simulink library "Lib_Piccolo"  (R2018b)
settings: Solver=VariableStepAuto  StartTime=0.0  StopTime=10.0  RelTol=1e-3
values from neighbouring files (symbols this model uses):
  AccelErrInt2Brakes = 0.15    [SimulationControlConfig16P.m]    (also in SimulationControlConfig16P_LEGACY.m; SimulationControlConfigTAILLESS.m = 0.2; SimulationControlConfigUTAIL.m = 0.2)
  AileronMax = 25    [SimulationControlConfig16P.m]    (also in SimulationControlConfig16P_LEGACY.m; SimulationControlConfigTAILLESS.m; SimulationControlConfigUTAIL.m)
  AileronPower = 0.00268    [SimulationControlConfig16P.m]    (also in SimulationControlConfig16P_LEGACY.m; SimulationControlConfigTAILLESS.m; SimulationControlConfigUTAIL.m)
  AileronSurfaceMax = 45    [SimulationControlConfig16P.m]    (also in SimulationControlConfig16P_LEGACY.m)
  AileronTrim = 0    [SimulationControlConfig16P.m]    (also in SimulationControlConfig16P_LEGACY.m; SimulationControlConfigTAILLESS.m; SimulationControlConfigUTAIL.m)
  Alt = 1000 + TerrainHeight    [SimulationStateConfig.m]
  AltCruise_m = testPlans(testIndx).terrainElevation * 0.3048 + 200    [SimulationControlConfig16P.m]    (also in SimulationControlConfigTAILLESS.m = 1083; SimulationControlConfigUTAIL.m = testPlans(testIndx).terrainElevation * 0.3048 + 152)
  AltitudeRate2PitchCmdIntegratorInit = 0.1    [SimulationControlPre.m]
  AltMax = 10000    [SimulationControlConfig16P.m]    (also in SimulationControlConfig16P_LEGACY.m; SimulationControlConfigTAILLESS.m; SimulationControlConfigUTAIL.m)
  AltMaxAccel = 1.25    [SimulationControlConfig16P.m]    (also in SimulationControlConfig16P_LEGACY.m = 0.9; SimulationControlConfigTAILLESS.m = 1.7; SimulationControlConfigUTAIL.m = 2)
  AltMin = 0    [SimulationControlConfig16P.m]    (also in SimulationControlConfig16P_LEGACY.m; SimulationControlConfigTAILLESS.m; SimulationControlConfigUTAIL.m)
  AltRateCmd2Pitch = 0.50    (= 0.5)    [SimulationControlConfig16P.m]    (also in SimulationControlConfig16P_LEGACY.m = 0.6; SimulationControlConfigTAILLESS.m = 0.2; SimulationControlConfigUTAIL.m = 0.3)
  AltRateError2Pitch = 0.40    (= 0.4)    [SimulationControlConfig16P.m]    (also in SimulationControlConfig16P_LEGACY.m; SimulationControlConfigTAILLESS.m = 0.55; SimulationControlConfigUTAIL.m = 0.55)
  AltRateErrorInt2Pitch = 0.50    (= 0.5)    [SimulationControlConfig16P.m]    (also in SimulationControlConfig16P_LEGACY.m = 0.45; SimulationControlConfigTAILLESS.m; SimulationControlConfigUTAIL.m = 0.75)
  AltRateLpfCutOff = 3    [SimulationControlConfig16P.m]    (also in SimulationControlConfig16P_LEGACY.m; SimulationControlConfigTAILLESS.m = 2; SimulationControlConfigUTAIL.m = 2)
  AutoNosegear2Rudder = 26    [SimulationControlConfig16P.m]    (also in SimulationControlConfig16P_LEGACY.m; SimulationControlConfigTAILLESS.m = 25.2; SimulationControlConfigUTAIL.m = 14)
  b = 5.54    [SimulationControlConfig16P.m]    (also in SimulationControlConfig16P_LEGACY.m; SimulationControlConfigTAILLESS.m = 2.37; SimulationControlConfigUTAIL.m = 2.37)
  Bank2AileronIntegratorInit = 0    [SimulationControlPre.m]
  BankMax_User = BankMax_User/180*pi    (= 0.523598775598)    [SimulationControlConfig16P.m]    (also in SimulationControlConfig16P_LEGACY.m; SimulationControlConfigTAILLESS.m = 0.610865238198; SimulationControlConfigUTAIL.m = 0.628318530718)
  baseLegFlaps = 20    [SimulationControlConfig16P.m]    (also in SimulationControlConfig16P_LEGACY.m = 0; SimulationControlConfigTAILLESS.m = 15; SimulationControlConfigUTAIL.m = 10)
  C = GeneticOpt.C    [SimulationCostFunction.m]
  c = Sw/b    (= 0.841696750903)    [SimulationControlConfig16P.m]    (also in SimulationControlConfig16P_LEGACY.m; SimulationControlConfigTAILLESS.m = 0.354008438819; SimulationControlConfigUTAIL.m = 0.354008438819)
  cell2WheelFactorMG = 5.98    [SimulationSensorConfig16P_LEGACY.m]
  cell2WheelFactorNG = 1    [SimulationSensorConfig16P_LEGACY.m]
  cellSatMaxMG = 15000    [SimulationSensorConfig16P.m]    (also in SimulationSensorConfig16P_LEGACY.m; SimulationSensorConfigTAILLESS7P.m; SimulationSensorConfigUTAIL7P.m)
  cellSatMaxNG = 1000    [SimulationSensorConfig16P.m]    (also in SimulationSensorConfig16P_LEGACY.m; SimulationSensorConfigTAILLESS7P.m; SimulationSensorConfigUTAIL7P.m)
  cellSatMinMG = -15000    [SimulationSensorConfig16P.m]    (also in SimulationSensorConfig16P_LEGACY.m; SimulationSensorConfigTAILLESS7P.m; SimulationSensorConfigUTAIL7P.m)
  cellSatMinNG = -1000    [SimulationSensorConfig16P.m]    (also in SimulationSensorConfig16P_LEGACY.m; SimulationSensorConfigTAILLESS7P.m; SimulationSensorConfigUTAIL7P.m)
  CL_Limit = CL_Max    (= 0.54)    [SimulationControlConfig16P.m]    (also in SimulationControlConfig16P_LEGACY.m; SimulationControlConfigTAILLESS.m; SimulationControlConfigUTAIL.m = 0.53)
  CL_Max = 0.54    [SimulationControlConfig16P.m]    (also in SimulationControlConfig16P_LEGACY.m; SimulationControlConfigTAILLESS.m; SimulationControlConfigUTAIL.m = 0.53)
  CL_Max_Nom = 0.465    [SimulationControlConfig16P.m]    (also in SimulationControlConfig16P_LEGACY.m; SimulationControlConfigTAILLESS.m = 0.39; SimulationControlConfigUTAIL.m)
  CL_Min = 0    [SimulationControlConfig16P.m]    (also in SimulationControlConfig16P_LEGACY.m; SimulationControlConfigTAILLESS.m; SimulationControlConfigUTAIL.m)
  ClimbMaxFraction = 0.35    [SimulationControlConfig16P.m]    (also in SimulationControlConfig16P_LEGACY.m = 0.24; SimulationControlConfigTAILLESS.m = 0.19; SimulationControlConfigUTAIL.m = 0.21)
  ClimboutMaxBank = 7.0    (= 7)    [SimulationControlConfig16P.m]    (also in SimulationControlConfig16P_LEGACY.m; SimulationControlConfigTAILLESS.m = 5; SimulationControlConfigUTAIL.m)
  ClimboutTimer = 7.0    (= 7)    [SimulationControlConfig16P.m]    (also in SimulationControlConfig16P_LEGACY.m; SimulationControlConfigTAILLESS.m; SimulationControlConfigUTAIL.m)
  dCl_per_dFlap = 0.005581818    [SimulationControlConfig16P.m]    (also in SimulationControlConfig16P_LEGACY.m = 0; SimulationControlConfigTAILLESS.m = 0; SimulationControlConfigUTAIL.m = 0)
  DecelerationCmd = 3.1    [SimulationControlConfig16P.m]    (also in SimulationControlConfig16P_LEGACY.m; SimulationControlConfigTAILLESS.m = 0.1; SimulationControlConfigUTAIL.m = 0.1)
  DeRotateLogicEndTimer = abs((NoseDownLimit_Deg-1)/DeRotateRamp_Dps)    [SimulationControlConfig16P.m]    (also in SimulationControlConfig16P_LEGACY.m; SimulationControlConfigTAILLESS.m; SimulationControlConfigUTAIL.m)
  DeRotateLogicHoldNoseUpTimer = 0.1    [SimulationControlConfig16P.m]    (also in SimulationControlConfig16P_LEGACY.m; SimulationControlConfigTAILLESS.m; SimulationControlConfigUTAIL.m)
  DeRotateLogicTimerTimeout = 2    [SimulationControlConfig16P.m]    (also in SimulationControlConfig16P_LEGACY.m; SimulationControlConfigTAILLESS.m; SimulationControlConfigUTAIL.m)
  DeRotateLowerCmdSaturation = 0    [SimulationControlConfig16P.m]    (also in SimulationControlConfig16P_LEGACY.m; SimulationControlConfigTAILLESS.m; SimulationControlConfigUTAIL.m)
  DeRotateRamp_Dps = 3    [SimulationControlConfig16P.m]    (also in SimulationControlConfig16P_LEGACY.m; SimulationControlConfigTAILLESS.m = 8; SimulationControlConfigUTAIL.m = 8)
  DeRotateUpperCmdSaturation = 7    [SimulationControlConfig16P.m]    (also in SimulationControlConfig16P_LEGACY.m; SimulationControlConfigTAILLESS.m; SimulationControlConfigUTAIL.m)
  DescentMaxFraction = 0.22    [SimulationControlConfig16P.m]    (also in SimulationControlConfig16P_LEGACY.m = 0.2; SimulationControlConfigTAILLESS.m = 0.17; SimulationControlConfigUTAIL.m = 0.17)
  DesktopSimTerrainOffset_m = 0.406    [SimulationAircraftConfig.m]
  downwindFlaps = 0    [SimulationControlConfig16P.m]    (also in SimulationControlConfig16P_LEGACY.m; SimulationControlConfigTAILLESS.m; SimulationControlConfigUTAIL.m)
  DP_init = 0.5*1.225*V_init^2    [SimulationControlConfig16P.m]    (also in SimulationControlConfig16P_LEGACY.m; SimulationControlConfigTAILLESS.m; SimulationControlConfigUTAIL.m)
  dscNoiseMG = 1    [SimulationSensorConfig16P_LEGACY.m]
  dscNoiseNG = 0.25    [SimulationSensorConfig16P_LEGACY.m]
  DSCnumBits = 24    [SimulationSensorConfig16P.m]    (also in SimulationSensorConfig16P_LEGACY.m; SimulationSensorConfigTAILLESS7P.m; SimulationSensorConfigUTAIL7P.m)
  DSCRangeMaxMG = 15000    [SimulationSensorConfig16P.m]    (also in SimulationSensorConfig16P_LEGACY.m; SimulationSensorConfigTAILLESS7P.m; SimulationSensorConfigUTAIL7P.m)
  DSCRangeMaxNG = 1000    [SimulationSensorConfig16P.m]    (also in SimulationSensorConfig16P_LEGACY.m; SimulationSensorConfigTAILLESS7P.m; SimulationSensorConfigUTAIL7P.m)
  DSCRangeMinMG = -15000    [SimulationSensorConfig16P.m]    (also in SimulationSensorConfig16P_LEGACY.m; SimulationSensorConfigTAILLESS7P.m; SimulationSensorConfigUTAIL7P.m)
  DSCRangeMinNG = -1000    [SimulationSensorConfig16P.m]    (also in SimulationSensorConfig16P_LEGACY.m; SimulationSensorConfigTAILLESS7P.m; SimulationSensorConfigUTAIL7P.m)
  dt = DLLSim.dt    [SimulationTimeStep.m]    (also in SimulationTrim.m = 0.02)
  EarlyTouchdownThreshold = 3.0    (= 3)    [SimulationControlConfig16P.m]    (also in SimulationControlConfig16P_LEGACY.m; SimulationControlConfigTAILLESS.m = 2.2; SimulationControlConfigUTAIL.m = 2.5)
  ElevatorDeflectionRate = 15    [SimulationControlConfig16P.m]    (also in SimulationControlConfig16P_LEGACY.m = 12; SimulationControlConfigTAILLESS.m = 10; SimulationControlConfigUTAIL.m = 12)
  ElevatorMax = 25    [SimulationControlConfig16P.m]    (also in SimulationControlConfig16P_LEGACY.m; SimulationControlConfigTAILLESS.m; SimulationControlConfigUTAIL.m)
  ElevatorPower = -0.002209    [SimulationControlConfig16P.m]    (also in SimulationControlConfig16P_LEGACY.m; SimulationControlConfigTAILLESS.m = -0.002956; SimulationControlConfigUTAIL.m = -0.00205983)
  ElevatorTrim = -3.5    [SimulationControlConfig16P.m]    (also in SimulationControlConfig16P_LEGACY.m; SimulationControlConfigTAILLESS.m = -6; SimulationControlConfigUTAIL.m = -8)
  elevonBias = 0    [SimulationControlConfig16P.m]    (also in SimulationControlConfig16P_LEGACY.m; SimulationControlConfigTAILLESS.m; SimulationControlConfigUTAIL.m)
  Enable_TAS_Protection = 0    [SimulationControlConfig16P.m]    (also in SimulationControlConfig16P_LEGACY.m; SimulationControlConfigTAILLESS.m; SimulationControlConfigUTAIL.m)
  EnableCrossTrackAbort = 1    [SimulationControlConfig16P.m]    (also in SimulationControlConfigTAILLESS.m; SimulationControlConfigUTAIL.m)
  EnergyBandwidth = 0.02    [SimulationControlConfig16P.m]    (also in SimulationControlConfig16P_LEGACY.m; SimulationControlConfigTAILLESS.m = 0.06; SimulationControlConfigUTAIL.m = 0.06)
  EngineLhFuelCut = 0    [SimulationAircraftConfig.m]
  EngineRhFuelCut = 0    [SimulationAircraftConfig.m]
  FastThrottleRate = 0.075    [SimulationControlConfig16P.m]    (also in SimulationControlConfig16P_LEGACY.m = 0.05; SimulationControlConfigTAILLESS.m = 0.1; SimulationControlConfigUTAIL.m = 0.1)
  FilterWarmUpTime = 2    [SimulationSensorConfig16P.m]    (also in SimulationSensorConfig16P_LEGACY.m; SimulationSensorConfigTAILLESS7P.m; SimulationSensorConfigUTAIL7P.m)
  finalApproachFlaps = 20    [SimulationControlConfig16P.m]    (also in SimulationControlConfig16P_LEGACY.m = 0; SimulationControlConfigTAILLESS.m = 22; SimulationControlConfigUTAIL.m = 10)
  FinalDescentSlope_Deg = testPlans(testIndx).descentSlope    [SimulationControlConfig16P.m]    (also in SimulationControlConfig16P_LEGACY.m; SimulationControlConfigTAILLESS.m; SimulationControlConfigUTAIL.m)
  flapMax = 0    [SimulationControlConfig16P.m]    (also in SimulationControlConfig16P_LEGACY.m; SimulationControlConfigTAILLESS.m; SimulationControlConfigUTAIL.m)
  flapRate = 7.5    [SimulationControlConfig16P.m]    (also in SimulationControlConfig16P_LEGACY.m; SimulationControlConfigTAILLESS.m = 6.6; SimulationControlConfigUTAIL.m)
  FlareHeight = 5    [SimulationControlConfig16P.m]    (also in SimulationControlConfig16P_LEGACY.m = 4.8; SimulationControlConfigTAILLESS.m = 2.5; SimulationControlConfigUTAIL.m = 2)
  FlareVerticalRate_mps = -0.4    [SimulationControlConfig16P.m]    (also in SimulationControlConfig16P_LEGACY.m = -0.5; SimulationControlConfigTAILLESS.m = -0.15; SimulationControlConfigUTAIL.m = -0.15)
  Fp_Aileron = 0.55*2*pi*RollRateLpfCutoff*dt    [SimulationControlConfig16P.m]    (also in SimulationControlConfig16P_LEGACY.m; SimulationControlConfigTAILLESS.m; SimulationControlConfigUTAIL.m)
  Fp_Alt = 0.55*AltBandwidth    (= 0.099)    [SimulationControlConfig16P.m]    (also in SimulationControlConfig16P_LEGACY.m; SimulationControlConfigTAILLESS.m = 0.587477826221; SimulationControlConfigUTAIL.m = 0.69115038379)
  Fp_AltRate = 0.55*2*pi*AltRateLpfCutOff*dt    [SimulationControlConfig16P.m]    (also in SimulationControlConfig16P_LEGACY.m; SimulationControlConfigTAILLESS.m; SimulationControlConfigUTAIL.m)
  Fp_Elevator = 0.55*2*pi*PitchRateLpfCutoff*dt    [SimulationControlConfig16P.m]    (also in SimulationControlConfig16P_LEGACY.m; SimulationControlConfigTAILLESS.m; SimulationControlConfigUTAIL.m)
  Fp_Energy = 0.55*2*pi*EnergyBandwidth    (= 0.069115038379)    [SimulationControlConfig16P.m]    (also in SimulationControlConfig16P_LEGACY.m; SimulationControlConfigTAILLESS.m = 0.207345115137; SimulationControlConfigUTAIL.m = 0.207345115137)
  Fp_Energy2 = 0.55*2*pi*EnergyBandwidth*dt    [SimulationControlConfig16P.m]    (also in SimulationControlConfig16P_LEGACY.m; SimulationControlConfigTAILLESS.m; SimulationControlConfigUTAIL.m)
  Fp_Pitch = 0.55*2*pi*PitchBandwidth    (= 2.76460153516)    [SimulationControlConfig16P.m]    (also in SimulationControlConfig16P_LEGACY.m = 3.11017672705; SimulationControlConfigTAILLESS.m = 3.80132711084; SimulationControlConfigUTAIL.m = 2.41902634326)
  Fp_Pitch_2 = 0.55*2*pi*PitchBandwidth*dt    [SimulationControlConfig16P.m]    (also in SimulationControlConfig16P_LEGACY.m; SimulationControlConfigTAILLESS.m; SimulationControlConfigUTAIL.m)
  Fp_Roll = RollBandwidth^2    (= 1)    [SimulationControlConfig16P.m]    (also in SimulationControlConfig16P_LEGACY.m = 1.44; SimulationControlConfigTAILLESS.m; SimulationControlConfigUTAIL.m)
  Fp_Rudder = 0.55*2*pi*YawRateLpfCutoff*dt    [SimulationControlConfig16P.m]    (also in SimulationControlConfig16P_LEGACY.m; SimulationControlConfigTAILLESS.m; SimulationControlConfigUTAIL.m)
  Fp_TAS = 0.55*2*pi*TASBandwidth    (= 0.103672557568)    [SimulationControlConfig16P.m]    (also in SimulationControlConfig16P_LEGACY.m; SimulationControlConfigTAILLESS.m = 0.172787595947; SimulationControlConfigUTAIL.m = 0.172787595947)
  Fp_TAS_Filter = 2*pi*TasLpfCutoff*dt    [SimulationControlConfig16P.m]    (also in SimulationControlConfig16P_LEGACY.m; SimulationControlConfigTAILLESS.m; SimulationControlConfigUTAIL.m)
  Fp_Turn = 0.55*2*pi*TurnErrLPFcutoff    (= 0.0345575191895)    [SimulationControlConfig16P.m]    (also in SimulationControlConfig16P_LEGACY.m; SimulationControlConfigTAILLESS.m = 0.172787595947; SimulationControlConfigUTAIL.m = 0.172787595947)
  Fp_TurnDerr = 0.55*2*pi*TurnDerivativeLPFcutoff    (= 0.0345575191895)    [SimulationControlConfig16P.m]    (also in SimulationControlConfig16P_LEGACY.m; SimulationControlConfigTAILLESS.m = 0.172787595947; SimulationControlConfigUTAIL.m = 0.172787595947)
  FTV = 3    [SimulationAircraftConfig.m]
  ftvStaticPositionError = 1/1.18    (= 0.847457627119)    [SimulationSensorConfig16P.m]    (also in SimulationSensorConfig16P_LEGACY.m; SimulationSensorConfigTAILLESS7P.m = 1; SimulationSensorConfigUTAIL7P.m = 1)
  g = 9.81    [SimulationStateConfig.m]
  GustSpd_Kts = testPlans(testIndx).gustSpd    [SimulationStateConfig.m]
  GustTriggerVal = testPlans(testIndx).gustTriggerVal    [SimulationStateConfig.m]
  HeadingErr2TurnRate = 0.5    [SimulationControlConfig16P.m]    (also in SimulationControlConfig16P_LEGACY.m; SimulationControlConfigTAILLESS.m; SimulationControlConfigUTAIL.m)
  HeadingErrDer2TurnRate = 0.3    [SimulationControlConfig16P.m]    (also in SimulationControlConfig16P_LEGACY.m; SimulationControlConfigTAILLESS.m; SimulationControlConfigUTAIL.m)
  IASbounce = IASstall*0.8    [SimulationControlPre.m]
  IAScruiseCMD = sqrt(2*m*9.81/(1.225*Sw*CL_cruise))    [SimulationControlConfig16P.m]    (also in SimulationControlConfig16P_LEGACY.m; SimulationControlConfigTAILLESS.m; SimulationControlConfigUTAIL.m)
  IASfinalCMD = 1.12 * IASmin    [SimulationControlConfig16P.m]    (also in SimulationControlConfig16P_LEGACY.m = 1.10 * IASmin; SimulationControlConfigTAILLESS.m = 1.10 * IASmin; SimulationControlConfigUTAIL.m = 1.15 * IASmin)
  IASflareCMD = IASstall    [SimulationControlConfig16P.m]    (also in SimulationControlConfig16P_LEGACY.m; SimulationControlConfigTAILLESS.m; SimulationControlConfigUTAIL.m)
  IASmax = 64    [SimulationControlConfig16P.m]    (also in SimulationControlConfig16P_LEGACY.m = 46; SimulationControlConfigTAILLESS.m = 38.58; SimulationControlConfigUTAIL.m = 35)
  IASmin = sqrt(2*m*9.81/(1.225*Sw*0.9*CL_Max_Nom))    [SimulationControlConfig16P.m]    (also in SimulationControlConfig16P_LEGACY.m; SimulationControlConfigTAILLESS.m; SimulationControlConfigUTAIL.m)
  IASshortCMD = IASstall    [SimulationControlConfig16P.m]    (also in SimulationControlConfig16P_LEGACY.m; SimulationControlConfigTAILLESS.m; SimulationControlConfigUTAIL.m)
  IASstall = sqrt(2*m*9.81/(1.225*Sw*CL_Max))    [SimulationControlConfig16P.m]    (also in SimulationControlConfig16P_LEGACY.m; SimulationControlConfigTAILLESS.m; SimulationControlConfigUTAIL.m)
  inFlight = 1    [SimulationControlConfig16P.m]    (also in SimulationControlConfigTAILLESS.m; SimulationControlConfigUTAIL.m)
  JetCatOffset = 5    [SimulationControlConfig16P.m]    (also in SimulationControlConfig16P_LEGACY.m)
  LaunchRollingElevator = -1.5    [SimulationControlConfig16P.m]    (also in SimulationControlConfig16P_LEGACY.m; SimulationControlConfigTAILLESS.m = 1; SimulationControlConfigUTAIL.m = 1)
  ldg_NosegearMax = 10    [SimulationControlConfig16P.m]    (also in SimulationControlConfig16P_LEGACY.m; SimulationControlConfigTAILLESS.m; SimulationControlConfigUTAIL.m)
  ldg_TrackVyErrInt2Nosegear = 0.1250    (= 0.125)    [SimulationControlConfig16P.m]    (also in SimulationControlConfig16P_LEGACY.m; SimulationControlConfigTAILLESS.m = 0.00714285714286; SimulationControlConfigUTAIL.m = 0.00714285714286)
  ldg_TrackVyErrPro2Nosegear = 0.35    [SimulationControlConfig16P.m]    (also in SimulationControlConfig16P_LEGACY.m; SimulationControlConfigTAILLESS.m = 0.0546666666667; SimulationControlConfigUTAIL.m = 0.0546666666667)
  ldg_TrackY2Vy = 0.07    [SimulationControlConfig16P.m]    (also in SimulationControlConfig16P_LEGACY.m; SimulationControlConfigTAILLESS.m = 0.17; SimulationControlConfigUTAIL.m = 0.17)
  ldg_Vy2NosegearScalingPower = 1.075    [SimulationControlConfig16P.m]    (also in SimulationControlConfig16P_LEGACY.m; SimulationControlConfigTAILLESS.m = 0.6; SimulationControlConfigUTAIL.m = 0.5)
  ldg_Y2VyScalingPower = 0.175    [SimulationControlConfig16P.m]    (also in SimulationControlConfig16P_LEGACY.m; SimulationControlConfigTAILLESS.m = 0; SimulationControlConfigUTAIL.m = 0)
  ldg_YawRate2Nosegear = 0.175    [SimulationControlConfig16P.m]    (also in SimulationControlConfig16P_LEGACY.m; SimulationControlConfigTAILLESS.m = 0.065; SimulationControlConfigUTAIL.m = 0.065)
  LiftSlope = 0.064285    [SimulationControlConfig16P.m]    (also in SimulationControlConfig16P_LEGACY.m; SimulationControlConfigTAILLESS.m = 0.058631; SimulationControlConfigUTAIL.m)
  LPFaileronInit = 0    [SimulationControlPre.m]
  LPFclestInit = 0    [SimulationControlPre.m]
  LPFenergyFFInit = 0    [SimulationControlPre.m]
  LPFtasInit = V_init + 2    [SimulationControlPre.m]
  LPFthrottleInit = ThrottleTrim    [SimulationControlPre.m]
  LPFturnErrInit = 0    [SimulationControlPre.m]
  ... (+115 more)
undefined symbols (not defined in the file or in its folder): abortFlag, alphaHPF, apmDelay, BRWNOUT, CRAWOR, CRAWUR, DiscIntNeverNeededParam, DLLSim, DLLSimStep, ECOMOR, ECOMUR, Fp_Tas, GustTrigger_HeightAgl_m, IPSTAT, LCINTEG, Ldg_Persist_Time, LOWER_FLAGS, MSG_ENABLE, NoiseStd, OLDVAL, OVERRIDE_ENABLE, OVERRIDE_VALUE, REBOOT, reversionEnable, revIASMax, revIASMin, revPitchMax, revPitchMin, revPitchRateMax, revRollMax, revRollRateMax, SAMPLE, SCALON, SensorModel, sigbuilder_block, Sim_Vx, Sim_Vy, Sim_Vz, Sim_Xpos, Sim_Ypos, Sim_Zpos, SYSOR, SYSUR, TARE, TEMPOR, TEMPUR, testIndx, testPlan, testPlans, Trim_piccoloInCmd, Trim_REFSI_FD_IN_nmodeCgShifterCmd_Ft, Trim_REFSI_FD_IN_nmodeFlapLhIBCmd_Deg, Trim_REFSI_FD_IN_nmodeFlapLhOBCmd_Deg, Trim_REFSI_FD_IN_nmodeFlapRhIBCmd_Deg, Trim_REFSI_FD_IN_nmodeFlapRhOBCmd_Deg, Trim_REFSI_FD_IN_nmodeSlatLhCmd_Deg, Trim_REFSI_FD_IN_nmodeSlatRhCmd_Deg, Trim_REFSI_FD_IN_nmodeSplrLhInbdCmd_Deg, Trim_REFSI_FD_IN_nmodeSplrLhOutbdCmd_Deg ... (+5)
libraries: simulink x866, aerolibconvert2 x60, $bdroot x52, aerolibatmos2 x5, dspswit3 x5, simulink_extras x4, dsparch4 x2, Lib_Piccolo_Alt x2, eeGeneralControl x1, dspindex x1
(part 18 of 44)

== system Lib_Piccolo/A//C Dynamics/DLLSimulation/Vector to Bus ==
  In1 : Inport
  BusCreator : BusCreator  Inputs=239
  Demux : Demux  Outputs=239
  Out1 : Outport
  wires:
  In1/1 -> Demux/1
  BusCreator/1 -> Out1/1
  Demux/1 -> BusCreator/1  "PresAltFt"
  Demux/2 -> BusCreator/2  "AlphaDeg"
  Demux/3 -> BusCreator/3  "BetaDeg"
  Demux/4 -> BusCreator/4  "GammaDeg"
  Demux/5 -> BusCreator/5  "CASKts"
  Demux/6 -> BusCreator/6  "PDps"
  Demux/7 -> BusCreator/7  "QDps"
  Demux/8 -> BusCreator/8  "RDps"
  Demux/9 -> BusCreator/9  "PhiDeg"
  Demux/10 -> BusCreator/10  "ThetaDeg"
  Demux/11 -> BusCreator/11  "PsiDeg"
  Demux/12 -> BusCreator/12  "TASKts"
  Demux/13 -> BusCreator/13  "HeightAGLFt"
  Demux/14 -> BusCreator/14  "XthrustLbs"
  Demux/15 -> BusCreator/15  "GrndContactLMG"
  Demux/16 -> BusCreator/16  "GrndContactNG"
  Demux/17 -> BusCreator/17  "GrndContactRMG"
  Demux/18 -> BusCreator/18  "DynPresPsf"
  Demux/19 -> BusCreator/19  "PAmbPsf"
  Demux/20 -> BusCreator/20  "XposnFt"
  Demux/21 -> BusCreator/21  "YposnFt"
  Demux/22 -> BusCreator/22  "ZposnFt"
  Demux/23 -> BusCreator/23  "NxG"
  Demux/24 -> BusCreator/24  "NyG"
  Demux/25 -> BusCreator/25  "NzG"
  Demux/26 -> BusCreator/26  "VEarthFtps_0"
  Demux/27 -> BusCreator/27  "VEarthFtps_1"
  Demux/28 -> BusCreator/28  "VEarthFtps_2"
  Demux/29 -> BusCreator/29  "LatitudeDeg"
  Demux/30 -> BusCreator/30  "LongitudeDeg"
  Demux/31 -> BusCreator/31  "ZgrndLhLbs"
  Demux/32 -> BusCreator/32  "ZgrndRhLbs"
  Demux/33 -> BusCreator/33  "ZgrndNgLbs"
  Demux/34 -> BusCreator/34  "Time"
  Demux/35 -> BusCreator/35  "WindUFtps"
  Demux/36 -> BusCreator/36  "WindVFtps"
  Demux/37 -> BusCreator/37  "WindWFtps"
  Demux/38 -> BusCreator/38  "AilLwrLhBDriveDeg"
  Demux/39 -> BusCreator/39  "AilUprLhBDriveDeg"
  Demux/40 -> BusCreator/40  "AilLwrRhBDriveDeg"
  Demux/41 -> BusCreator/41  "AilUprRhBDriveDeg"
  Demux/42 -> BusCreator/42  "ElvLhOBBDriveDeg"
  Demux/43 -> BusCreator/43  "ElvLhIBBDriveDeg"
  Demux/44 -> BusCreator/44  "ElvRhOBBDriveDeg"
  Demux/45 -> BusCreator/45  "ElvRhIBBDriveDeg"
  Demux/46 -> BusCreator/46  "RudPylLhBDriveDeg"
  Demux/47 -> BusCreator/47  "RudUTailLhBDriveDeg"
  Demux/48 -> BusCreator/48  "RudWingletLhBDriveDeg"
  Demux/49 -> BusCreator/49  "ElvUTailLhBDriveDeg"
  Demux/50 -> BusCreator/50  "ElvUTailRhBDriveDeg"
  Demux/51 -> BusCreator/51  "RudPylRhBDriveDeg"
  Demux/52 -> BusCreator/52  "RudUTailRhBDriveDeg"
  Demux/53 -> BusCreator/53  "RudWingletRhBDriveDeg"
  Demux/54 -> BusCreator/54  "AftFlapBDriveDeg"
  Demux/55 -> BusCreator/55  "NWBDriveDeg"
  Demux/56 -> BusCreator/56  "XcgPctMAC"
  Demux/57 -> BusCreator/57  "IxxLbsInch2"
  Demux/58 -> BusCreator/58  "IyyLbsInch2"
  Demux/59 -> BusCreator/59  "IzzLbsInch2"
  Demux/60 -> BusCreator/60  "IxzLbsInch2"
  Demux/61 -> BusCreator/61  "REFSI_FD_OUT_PIC_dynPres_Pa"
  Demux/62 -> BusCreator/62  "REFSI_FD_OUT_PIC_TAmb_C"
  Demux/63 -> BusCreator/63  "REFSI_FD_OUT_PIC_PAmb_Pa"
  Demux/64 -> BusCreator/64  "REFSI_FD_OUT_PIC_rollRate_Dps"
  Demux/65 -> BusCreator/65  "REFSI_FD_OUT_PIC_pitchRate_Dps"
  Demux/66 -> BusCreator/66  "REFSI_FD_OUT_PIC_yawRate_Dps"
  Demux/67 -> BusCreator/67  "REFSI_FD_OUT_PIC_accelXDir_Mps2"
  Demux/68 -> BusCreator/68  "REFSI_FD_OUT_PIC_accelYDir_Mps2"
  Demux/69 -> BusCreator/69  "REFSI_FD_OUT_PIC_accelZDir_Mps2"
  Demux/70 -> BusCreator/70  "REFSI_FD_OUT_PIC_GPSUbloxLatitudeDeg"
  Demux/71 -> BusCreator/71  "REFSI_FD_OUT_PIC_GPSUbloxLongitudeDeg"
  Demux/72 -> BusCreator/72  "REFSI_FD_OUT_PIC_GPSUbloxHeight_m"
  Demux/73 -> BusCreator/73  "REFSI_FD_OUT_PIC_vEarthXUblox_Mps"
  Demux/74 -> BusCreator/74  "REFSI_FD_OUT_PIC_vEarthYUblox_Mps"
  Demux/75 -> BusCreator/75  "REFSI_FD_OUT_PIC_vEarthZUblox_Mps"
  Demux/76 -> BusCreator/76  "REFSI_FD_OUT_PIC_GPSNovAftLatitudeDeg"
  Demux/77 -> BusCreator/77  "REFSI_FD_OUT_PIC_GPSNovAftLongitudeDeg"
  Demux/78 -> BusCreator/78  "REFSI_FD_OUT_PIC_GPSNovAftHeight_m"
  Demux/79 -> BusCreator/79  "REFSI_FD_OUT_PIC_vEarthXNovAft_Mps"
  Demux/80 -> BusCreator/80  "REFSI_FD_OUT_PIC_vEarthYNovAft_Mps"
  Demux/81 -> BusCreator/81  "REFSI_FD_OUT_PIC_vEarthZNovAft_Mps"
  Demux/82 -> BusCreator/82  "ismCas_Kt"
  Demux/83 -> BusCreator/83  "ismTas_Kt"
  Demux/84 -> BusCreator/84  "ismPresAlt_Ft"
  Demux/85 -> BusCreator/85  "ismDynPres_Psf"
  Demux/86 -> BusCreator/86  "ismAoa_Deg"
  Demux/87 -> BusCreator/87  "ismAos_Deg"
  Demux/88 -> BusCreator/88  "speedIncrementImuXRaw_Mps"
  Demux/89 -> BusCreator/89  "speedIncrementImuYRaw_Mps"
  Demux/90 -> BusCreator/90  "speedIncrementImuZRaw_Mps"
  Demux/91 -> BusCreator/91  "rollIncrementRaw_Deg"
  Demux/92 -> BusCreator/92  "pitchIncrementRaw_Deg"
  Demux/93 -> BusCreator/93  "yawIncrementRaw_Deg"
  Demux/94 -> BusCreator/94  "latitudeRaw_Rad"
  Demux/95 -> BusCreator/95  "longitudeRaw_Rad"
  Demux/96 -> BusCreator/96  "heightRaw_M"
  Demux/97 -> BusCreator/97  "speedGpsIneNavXRaw_Mps"
  Demux/98 -> BusCreator/98  "speedGpsIneNavYRaw_Mps"
  Demux/99 -> BusCreator/99  "speedGpsIneNavZRaw_Mps"
  Demux/100 -> BusCreator/100  "isGpsMeasurementValid"
  Demux/101 -> BusCreator/101  "gpsDelay_s"
  Demux/102 -> BusCreator/102  "latitudeStandardDeviation_M"
  Demux/103 -> BusCreator/103  "longitudeStandardDeviation_M"
  Demux/104 -> BusCreator/104  "heightStandardDeviation_M"
  Demux/105 -> BusCreator/105  "speedXStandardDeviation_Mps"
  Demux/106 -> BusCreator/106  "speedYStandardDeviation_Mps"
  Demux/107 -> BusCreator/107  "speedZStandardDeviation_Mps"
  Demux/108 -> BusCreator/108  "gpsMode"
  Demux/109 -> BusCreator/109  "latitudePiccolo_Rad"
  Demux/110 -> BusCreator/110  "longitudePiccolo_Rad"
  Demux/111 -> BusCreator/111  "heightPiccolo_M"
  Demux/112 -> BusCreator/112  "speedGpsIneNavXPiccolo_Mps"
  Demux/113 -> BusCreator/113  "speedGpsIneNavYPiccolo_Mps"
  Demux/114 -> BusCreator/114  "speedGpsIneNavZPiccolo_Mps"
  Demux/115 -> BusCreator/115  "rollAttitudePiccolo_Deg"
  Demux/116 -> BusCreator/116  "pitchAttitudePiccolo_Deg"
  Demux/117 -> BusCreator/117  "yawAttitudePiccolo_Deg"
  Demux/118 -> BusCreator/118  "rollRatePiccolo_Dps"
  Demux/119 -> BusCreator/119  "pitchRatePiccolo_Dps"
  Demux/120 -> BusCreator/120  "yawRatePiccolo_Dps"
  Demux/121 -> BusCreator/121  "nxPiccolo"
  Demux/122 -> BusCreator/122  "nyPiccolo"
  Demux/123 -> BusCreator/123  "nzPiccolo"
  Demux/124 -> BusCreator/124  "piccoloDelay_s"
  Demux/125 -> BusCreator/125  "ismTLALh_Deg"
  Demux/126 -> BusCreator/126  "ismTLARh_Deg"
  Demux/127 -> BusCreator/127  "REFSI_AC_OUT_nmodeRudLhWingCmd_Deg"
  Demux/128 -> BusCreator/128  "REFSI_AC_OUT_nmodeAilLhLowerCmd_Deg"
  Demux/129 -> BusCreator/129  "REFSI_AC_OUT_nmodeAilLhUpperCmd_Deg"
  Demux/130 -> BusCreator/130  "REFSI_AC_OUT_nmodeElvLhOutbdCmd_Deg"
  Demux/131 -> BusCreator/131  "REFSI_AC_OUT_nmodeElvLhInbdCmd_Deg"
  Demux/132 -> BusCreator/132  "REFSI_AC_OUT_nmodeRudLhPylonCmd_Deg"
  Demux/133 -> BusCreator/133  "REFSI_AC_OUT_nmodeRudLhUTailCmd_Deg"
  Demux/134 -> BusCreator/134  "REFSI_AC_OUT_nmodeElvLhUTailCmd_Deg"
  Demux/135 -> BusCreator/135  "REFSI_AC_OUT_nmodeAftFlapCmd_Deg"
  Demux/136 -> BusCreator/136  "REFSI_AC_OUT_nmodeElvRhUTailCmd_Deg"
  Demux/137 -> BusCreator/137  "REFSI_AC_OUT_nmodeRudRhUTailCmd_Deg"
  Demux/138 -> BusCreator/138  "REFSI_AC_OUT_nmodeRudRhPylonCmd_Deg"
  Demux/139 -> BusCreator/139  "REFSI_AC_OUT_nmodeElvRhInbdCmd_Deg"
  Demux/140 -> BusCreator/140  "REFSI_AC_OUT_nmodeElvRhOutbdCmd_Deg"
  Demux/141 -> BusCreator/141  "REFSI_AC_OUT_nmodeAilRhUpperCmd_Deg"
  Demux/142 -> BusCreator/142  "REFSI_AC_OUT_nmodeAilRhLowerCmd_Deg"
  Demux/143 -> BusCreator/143  "REFSI_AC_OUT_nmodeRudRhWingCmd_Deg"
  Demux/144 -> BusCreator/144  "AilLwrLhLoadPct"
  Demux/145 -> BusCreator/145  "AilUprLhLoadPct"
  Demux/146 -> BusCreator/146  "AilLwrRhLoadPct"
  Demux/147 -> BusCreator/147  "AilUprRhLoadPct"
  Demux/148 -> BusCreator/148  "ElvLhOBLoadPct"
  Demux/149 -> BusCreator/149  "ElvLhIBLoadPct"
  Demux/150 -> BusCreator/150  "ElvRhOBLoadPct"
  Demux/151 -> BusCreator/151  "ElvRhIBLoadPct"
  Demux/152 -> BusCreator/152  "RudPylLhLoadPct"
  Demux/153 -> BusCreator/153  "RudUTailLhLoadPct"
  Demux/154 -> BusCreator/154  "RudWingletLhLoadPct"
  Demux/155 -> BusCreator/155  "ElvUTailLhLoadPct"
  Demux/156 -> BusCreator/156  "ElvUTailRhLoadPct"
  Demux/157 -> BusCreator/157  "RudPylRhLoadPct"
  Demux/158 -> BusCreator/158  "RudUTailRhLoadPct"
  Demux/159 -> BusCreator/159  "RudWingletRhLoadPct"
  Demux/160 -> BusCreator/160  "AftFlapLoadPct"
  Demux/161 -> BusCreator/161  "HMRudWgltLhInLb"
  Demux/162 -> BusCreator/162  "HMAilLwrLhInLb"
  Demux/163 -> BusCreator/163  "HMAilUprLhInLb"
  Demux/164 -> BusCreator/164  "HMElevonOBLhInLb"
  Demux/165 -> BusCreator/165  "HMElevonIBLhInLb"
  Demux/166 -> BusCreator/166  "HMRudPylLhInLb"
  Demux/167 -> BusCreator/167  "HMElvLhInLb"
  Demux/168 -> BusCreator/168  "HMRudUtailLhInLb"
  Demux/169 -> BusCreator/169  "HMAftFlapInLb"
  Demux/170 -> BusCreator/170  "HMRudUtailRhInLb"
  Demux/171 -> BusCreator/171  "HMElvRhInLb"
  Demux/172 -> BusCreator/172  "HMRudPylRhInLb"
  Demux/173 -> BusCreator/173  "HMElevonIBRhInLb"
  Demux/174 -> BusCreator/174  "HMElevonOBRhInLb"
  Demux/175 -> BusCreator/175  "HMAilUprRhInLb"
  Demux/176 -> BusCreator/176  "HMAilLwrRhInLb"
  Demux/177 -> BusCreator/177  "HMRudWgltRhInLb"
  Demux/178 -> BusCreator/178  "CgShifterPosn_Ft"
  Demux/179 -> BusCreator/179  "N1PctLhCmd"
  Demux/180 -> BusCreator/180  "N1PctRhCmd"
  Demux/181 -> BusCreator/181  "FlapLhOBBDriveDeg"
  Demux/182 -> BusCreator/182  "FlapLhIBBDriveDeg"
  Demux/183 -> BusCreator/183  "SlatLhBDriveDeg"
  Demux/184 -> BusCreator/184  "SlatRhBDriveDeg"
  Demux/185 -> BusCreator/185  "FlapRhOBBDriveDeg"
  Demux/186 -> BusCreator/186  "FlapRhIBBDriveDeg"
  Demux/187 -> BusCreator/187  "BrakeLh"
  Demux/188 -> BusCreator/188  "BrakeRh"
  Demux/189 -> BusCreator/189  "MFS1LhBDriveDeg"
  Demux/190 -> BusCreator/190  "GrndSplrLhBDriveDeg"
  Demux/191 -> BusCreator/191  "GrndSplrRhBDriveDeg"
  Demux/192 -> BusCreator/192  "MFS1RhBDriveDeg"
  Demux/193 -> BusCreator/193  "REFSI_FD_OUT_PIC_GPSNovFwdLatitudeDeg"
  Demux/194 -> BusCreator/194  "REFSI_FD_OUT_PIC_GPSNovFwdLongitudeDeg"
  Demux/195 -> BusCreator/195  "REFSI_FD_OUT_PIC_GPSNovFwdHeight_m"
  Demux/196 -> BusCreator/196  "REFSI_FD_OUT_PIC_vEarthXNovFwd_Mps"
  Demux/197 -> BusCreator/197  "REFSI_FD_OUT_PIC_vEarthYNovFwd_Mps"
  Demux/198 -> BusCreator/198  "REFSI_FD_OUT_PIC_vEarthZNovFwd_Mps"
  Demux/199 -> BusCreator/199  "ismRollAccel_Dps2"
  Demux/200 -> BusCreator/200  "ismPitchAccel_Dps2"
  Demux/201 -> BusCreator/201  "ismYawAccel_Dps2"
  Demux/202 -> BusCreator/202  "ismFuelBurnRateLh_Lpm"
  Demux/203 -> BusCreator/203  "ismFuelBurnRateRh_Lpm"
  Demux/204 -> BusCreator/204  "ismFuelBurntLh_Lbs"
  Demux/205 -> BusCreator/205  "ismFuelBurntRh_Lbs"
  Demux/206 -> BusCreator/206  "ismN1Lh_Pct"
  Demux/207 -> BusCreator/207  "ismN1Rh_Pct"
  Demux/208 -> BusCreator/208  "ismRudWingletLhPosn_Deg"
  Demux/209 -> BusCreator/209  "ismAilLwrLhPosn_Deg"
  Demux/210 -> BusCreator/210  "ismAilUprLhPosn_Deg"
  Demux/211 -> BusCreator/211  "ismElvLhOBPosn_Deg"
  Demux/212 -> BusCreator/212  "ismElvLhIBPosn_Deg"
  Demux/213 -> BusCreator/213  "ismRudPylLhPosn_Deg"
  Demux/214 -> BusCreator/214  "ismRudUTailLhPosn_Deg"
  Demux/215 -> BusCreator/215  "ismElvUTailLhPosn_Deg"
  Demux/216 -> BusCreator/216  "ismElvUTailRhPosn_Deg"
  Demux/217 -> BusCreator/217  "ismRudUTailRhPosn_Deg"
  Demux/218 -> BusCreator/218  "ismRudPylRhPosn_Deg"
  Demux/219 -> BusCreator/219  "ismElvRhIBPosn_Deg"
  Demux/220 -> BusCreator/220  "ismElvRhOBPosn_Deg"
  Demux/221 -> BusCreator/221  "ismAilUprRhPosn_Deg"
  Demux/222 -> BusCreator/222  "ismAilLwrRhPosn_Deg"
  Demux/223 -> BusCreator/223  "ismRudWingletRhPosn_Deg"
  Demux/224 -> BusCreator/224  "ismFlapLhIBPosn_Deg"
  Demux/225 -> BusCreator/225  "ismFlapRhIBPosn_Deg"
  Demux/226 -> BusCreator/226  "ismFlapLhOBPosn_Deg"
  Demux/227 -> BusCreator/227  "ismFlapRhOBPosn_Deg"
  Demux/228 -> BusCreator/228  "ismSlatLhPosn_Deg"
  Demux/229 -> BusCreator/229  "ismSlatRhPosn_Deg"
  Demux/230 -> BusCreator/230  "ismAftFlapPosn_Deg"
  Demux/231 -> BusCreator/231  "ismNoseGearPosn_Deg"
  Demux/232 -> BusCreator/232  "ismStabPosn_Deg"
  Demux/233 -> BusCreator/233  "ismSplrLhOutbdPosn_Deg"
  Demux/234 -> BusCreator/234  "ismSplrLhInbdPosn_Deg"
  Demux/235 -> BusCreator/235  "ismSplrRhInbdPosn_Deg"
  Demux/236 -> BusCreator/236  "ismSplrRhOutbdPosn_Deg"
  Demux/237 -> BusCreator/237  "ismCgShifterPosn_Ft"
  Demux/238 -> BusCreator/238  "ismWeightOnWheel"
  Demux/239 -> BusCreator/239  "ismHeightAboveGround_Ft"

== system Lib_Piccolo/A//C Dynamics/DLLSimulation/Vector to Bus v16_ ==
  In1 : Inport
  Vector to Bus 16P5 - v16 : Subsystem  VariantControl="modelScale == \"16P5\""  mask{Nsigs=DLLSim.nOuputs}
      mask prompts: Nsigs "Signal Length"
  Vector to Bus 7P - v16 : Subsystem  VariantControl="modelScale == \"7P\""  mask{Nsigs=DLLSim.nOuputs}
      mask prompts: Nsigs "Signal Length"
  Out1 : Outport

== system Lib_Piccolo/A//C Dynamics/Gust Wind Input1/Gust Wind Model ==
  BA Sim Input IN : Inport
  Trigger : Inport  Port=2
  Bus Assignment : BusAssignment  AssignedSignals=RefWindSpdKts
  Constant : Constant
  Gust Models : Subsystem  Variant=on
  Latch : Subsystem
  Sum : Sum  Inputs=++|
  Timer : Subsystem  mask{period=3}
      mask prompts: period "Period [s]"
  Wind Bias : Constant  Value=WindSpd_Kts
  BA Sim Input OUT : Outport
  wires:
  BA Sim Input IN/1 -> Bus Assignment/1
  Bus Assignment/1 -> BA Sim Input OUT/1
  Wind Bias/1 -> Sum/1
  Gust Models/1(gustSpdOut_kts) -> Sum/2
  Sum/1 -> Bus Assignment/2  "Sim.WindSpdKts"
  Timer/1(timeOut_s) -> Gust Models/1(timeIn_s)
  Latch/1(Q_Latched) -> Timer/1(Run/!Reset)
  Trigger/1 -> Latch/1(D)
  Constant/1 -> Latch/2(Enable/!Rst)

== system Lib_Piccolo/A//C Dynamics/Gust Wind Input1/No Gust ==
  BA Sim Input IN : Inport
  Trigger : Inport  Port=2
  Terminator : Terminator
  Terminator1 : Terminator
  Wind Bias : Constant  Value=WindSpd_Kts
  BA Sim Input OUT : Outport
  wires:
  BA Sim Input IN/1 -> BA Sim Input OUT/1
  Trigger/1 -> Terminator/1
  Wind Bias/1 -> Terminator1/1  "Sim.WindSpdKts"

== system Lib_Piccolo/A//C Dynamics/SIM Exit Conditions/Timer ==
  Enable/!Rst : Inport
  Compare To Constant1 : simulink/Logic and Bit Operations/Compare To Constant  relop=>  const=0  OutDataTypeStr=uint8
  Compare To Constant2 : simulink/Logic and Bit Operations/Compare To Constant  relop=>=  const=period  OutDataTypeStr=uint8
  Compare To Constant3 : simulink/Logic and Bit Operations/Compare To Constant  relop===  const=0  OutDataTypeStr=boolean
  Discrete-Time Integrator : DiscreteIntegrator  ExternalReset=level  SampleTime=-1  OutDataTypeStr=double  ICPrevOutput=DiscIntNeverNeededParam  ICPrevScaledInput=DiscIntNeverNeededParam
  Expired : Outport
  wires:
  Compare To Constant1/1 -> Discrete-Time Integrator/1
  Compare To Constant2/1 -> Expired/1
  Discrete-Time Integrator/1 -> Compare To Constant2/1
  Enable/!Rst/1 -> Compare To Constant1/1, Compare To Constant3/1
  Compare To Constant3/1 -> Discrete-Time Integrator/2

== system Lib_Piccolo/A//C Dynamics/Simulated Piccolo Commands/Signal Builder2 ==
  Demux : Demux  Tag=STV Demux
  FromWs : FromWorkspace  Tag=STV FromWs  VariableName=tuvar  SampleTime=0
      SigBuilderData=|
      | common.afterFinalStr = 'Extrapolate'
      | common.sampleTime = 0
      | dataSet.timeRange = [0 50]
      | dataSet.name = 'Group 1'
      | sbobj.Groups.Name = 'Group 1'
      | sbobj.Groups.Signals(1).Name = 'Signal 3'
      | sbobj.Groups.Signals(1).XData = [0 1 1 50]
      | sbobj.Groups.Signals(1).YData = [0 0 -1 -1]
      | sbobj.Groups.Signals(2).Name = 'Signal 1'
      | sbobj.Groups.Signals(2).XData = [0 20 20 30 30 50]
      | sbobj.Groups.Signals(2).YData = [0 0 0.4 0.4 0 0]
      | sbobj.Groups.Signals(3).Name = 'Signal 2'
      | sbobj.Groups.Signals(3).XData = [0 0.5 0.5 50]
      | sbobj.Groups.Signals(3).YData = [1 1 0 0]
      | sbobj.Groups.Signals(4).Name = 'Signal 4'
      | sbobj.Groups.Signals(4).XData = [0 0.1 0.1 50]
      | sbobj.Groups.Signals(4).YData = [1 1 0 0]
      | sbobj.Groups.TimeRange = [0 50]
  Signal 3 : Outport  Tag=STV Outport
  Signal 1 : Outport  Tag=STV Outport  Port=2
  Signal 2 : Outport  Tag=STV Outport  Port=3
  Signal 4 : Outport  Tag=STV Outport  Port=4
  wires:
  FromWs/1 -> Demux/1
  Demux/1 -> Signal 3/1
  Demux/2 -> Signal 1/1
  Demux/3 -> Signal 2/1
  Demux/4 -> Signal 4/1

== system Lib_Piccolo/A//C Dynamics/Simulated Piccolo Commands/Subsystem ==
  In1 : Inport
  Add : Sum  Inputs=++|
  Bus Selector6 : BusSelector  OutputSignals=REFSI_AC_OUT_nmodeRudLhWingCmd_Deg  OutputAsBus=on
  Product : Product
  CLAWS_RudWingletLhCmdDeg : Outport
  wires:
  Add/1 -> CLAWS_RudWingletLhCmdDeg/1  "REFSI_FD_IN_nmodeRudLhWingCmd_Deg"
  [CLAWsCommands] -> Bus Selector6/1
  In1/1 -> Add/2
  Bus Selector6/1 -> Product/2
  Product/1 -> Add/1
  [CLAWsOn] -> Product/1

== system Lib_Piccolo/A//C Dynamics/Simulated Piccolo Commands/Subsystem1 ==
  In1 : Inport
  Add : Sum  Inputs=++|
  Bus Selector6 : BusSelector  OutputSignals=REFSI_AC_OUT_nmodeAilLhLowerCmd_Deg  OutputAsBus=on
  Product : Product
  CLAWS_AilLwrLhCmdDeg : Outport
  wires:
  [CLAWsOn] -> Product/1
  Product/1 -> Add/1
  Bus Selector6/1 -> Product/2
  In1/1 -> Add/2
  [CLAWsCommands] -> Bus Selector6/1
  Add/1 -> CLAWS_AilLwrLhCmdDeg/1  "REFSI_FD_IN_nmodeAilLhLowerCmd_Deg"

== system Lib_Piccolo/A//C Dynamics/Simulated Piccolo Commands/Subsystem10 ==
  In1 : Inport
  Add : Sum  Inputs=++|
  Bus Selector6 : BusSelector  OutputSignals=REFSI_AC_OUT_nmodeRudRhUTailCmd_Deg
  Product : Product
  CLAWS_RudUTailRhCmdDeg : Outport
  wires:
  Add/1 -> CLAWS_RudUTailRhCmdDeg/1  "REFSI_FD_IN_nmodeRudRhUTailCmd_Deg"
  [CLAWsCommands] -> Bus Selector6/1
  In1/1 -> Add/2
  Bus Selector6/1 -> Product/2  "<REFSI_AC_OUT_nmodeRudRhUTailCmd_Deg>"
  Product/1 -> Add/1
  [CLAWsOn] -> Product/1

== system Lib_Piccolo/A//C Dynamics/Simulated Piccolo Commands/Subsystem11 ==
  In1 : Inport
  Add : Sum  Inputs=++|
  Bus Selector6 : BusSelector  OutputSignals=REFSI_AC_OUT_nmodeRudRhPylonCmd_Deg
  Product : Product
  CLAWS_RudPylRhCmdDeg : Outport
  wires:
  [CLAWsOn] -> Product/1
  Product/1 -> Add/1
  Bus Selector6/1 -> Product/2  "<REFSI_AC_OUT_nmodeRudRhPylonCmd_Deg>"
  In1/1 -> Add/2
  [CLAWsCommands] -> Bus Selector6/1
  Add/1 -> CLAWS_RudPylRhCmdDeg/1  "REFSI_FD_IN_nmodeRudRhPylonCmd_Deg"

== system Lib_Piccolo/A//C Dynamics/Simulated Piccolo Commands/Subsystem12 ==
  In1 : Inport
  Add : Sum  Inputs=++|
  Bus Selector6 : BusSelector  OutputSignals=REFSI_AC_OUT_nmodeElvRhInbdCmd_Deg
  Product : Product
  CLAWS_ElvRhIBCmdDeg : Outport
  wires:
  Add/1 -> CLAWS_ElvRhIBCmdDeg/1  "REFSI_FD_IN_nmodeElvRhInbdCmd_Deg"
  [CLAWsCommands] -> Bus Selector6/1
  In1/1 -> Add/2
  Bus Selector6/1 -> Product/2  "<REFSI_AC_OUT_nmodeElvRhInbdCmd_Deg>"
  Product/1 -> Add/1
  [CLAWsOn] -> Product/1

== system Lib_Piccolo/A//C Dynamics/Simulated Piccolo Commands/Subsystem13 ==
  In1 : Inport
  Add : Sum  Inputs=++|
  Bus Selector6 : BusSelector  OutputSignals=REFSI_AC_OUT_nmodeElvRhOutbdCmd_Deg
  Product : Product
  CLAWS_ElvRhOBCmdDeg : Outport
  wires:
  [CLAWsOn] -> Product/1
  Product/1 -> Add/1
  Bus Selector6/1 -> Product/2  "<REFSI_AC_OUT_nmodeElvRhOutbdCmd_Deg>"
  In1/1 -> Add/2
  [CLAWsCommands] -> Bus Selector6/1
  Add/1 -> CLAWS_ElvRhOBCmdDeg/1  "REFSI_FD_IN_nmodeElvRhOutbdCmd_Deg"

== system Lib_Piccolo/A//C Dynamics/Simulated Piccolo Commands/Subsystem14 ==
  In1 : Inport
  Add : Sum  Inputs=++|
  Bus Selector6 : BusSelector  OutputSignals=REFSI_AC_OUT_nmodeAilRhUpperCmd_Deg
  Product : Product
  CLAWS_AilUprRhCmdDeg : Outport
  wires:
  Add/1 -> CLAWS_AilUprRhCmdDeg/1  "REFSI_FD_IN_nmodeAilRhUpperCmd_Deg"
  [CLAWsCommands] -> Bus Selector6/1
  In1/1 -> Add/2
  Bus Selector6/1 -> Product/2  "<REFSI_AC_OUT_nmodeAilRhUpperCmd_Deg>"
  Product/1 -> Add/1
  [CLAWsOn] -> Product/1

== system Lib_Piccolo/A//C Dynamics/Simulated Piccolo Commands/Subsystem15 ==
  In1 : Inport
  Add : Sum  Inputs=++|
  Bus Selector6 : BusSelector  OutputSignals=REFSI_AC_OUT_nmodeAilRhLowerCmd_Deg
  Product : Product
  CLAWS_AilLwrRhCmdDeg : Outport
  wires:
  [CLAWsOn] -> Product/1
  Product/1 -> Add/1
  Bus Selector6/1 -> Product/2  "<REFSI_AC_OUT_nmodeAilRhLowerCmd_Deg>"
  In1/1 -> Add/2
  [CLAWsCommands] -> Bus Selector6/1
  Add/1 -> CLAWS_AilLwrRhCmdDeg/1  "REFSI_FD_IN_nmodeAilRhLowerCmd_Deg"

== system Lib_Piccolo/A//C Dynamics/Simulated Piccolo Commands/Subsystem16 ==
  In1 : Inport
  Add : Sum  Inputs=++|
  Bus Selector6 : BusSelector  OutputSignals=REFSI_AC_OUT_nmodeRudRhWingCmd_Deg
  Product : Product
  CLAWS_RudWingletRhCmdDeg : Outport
  wires:
  Add/1 -> CLAWS_RudWingletRhCmdDeg/1  "REFSI_FD_IN_nmodeRudRhWingCmd_Deg"
  [CLAWsCommands] -> Bus Selector6/1
  In1/1 -> Add/2
  Bus Selector6/1 -> Product/2  "<REFSI_AC_OUT_nmodeRudRhWingCmd_Deg>"
  Product/1 -> Add/1
  [CLAWsOn] -> Product/1

== system Lib_Piccolo/A//C Dynamics/Simulated Piccolo Commands/Subsystem2 ==
  In1 : Inport
  Add : Sum  Inputs=++|
  Bus Selector6 : BusSelector  OutputSignals=REFSI_AC_OUT_nmodeAilLhUpperCmd_Deg  OutputAsBus=on
  Product : Product
  CLAWS_AilUprLhCmdDeg : Outport
  wires:
  Add/1 -> CLAWS_AilUprLhCmdDeg/1  "REFSI_FD_IN_nmodeAilLhUpperCmd_Deg"
  [CLAWsCommands] -> Bus Selector6/1
  In1/1 -> Add/2
  Bus Selector6/1 -> Product/2
  Product/1 -> Add/1
  [CLAWsOn] -> Product/1

== system Lib_Piccolo/A//C Dynamics/Simulated Piccolo Commands/Subsystem3 ==
  In1 : Inport
  Add : Sum  Inputs=++|
  Bus Selector6 : BusSelector  OutputSignals=REFSI_AC_OUT_nmodeElvLhOutbdCmd_Deg  OutputAsBus=on
  Product : Product
  CLAWS_ElvLhOBCmdDeg : Outport
  wires:
  [CLAWsOn] -> Product/1
  Product/1 -> Add/1
  Bus Selector6/1 -> Product/2
  In1/1 -> Add/2
  [CLAWsCommands] -> Bus Selector6/1
  Add/1 -> CLAWS_ElvLhOBCmdDeg/1  "REFSI_FD_IN_nmodeElvLhOutbdCmd_Deg"

== system Lib_Piccolo/A//C Dynamics/Simulated Piccolo Commands/Subsystem4 ==
  In1 : Inport
  Add : Sum  Inputs=++|
  Bus Selector6 : BusSelector  OutputSignals=REFSI_AC_OUT_nmodeElvLhInbdCmd_Deg  OutputAsBus=on
  Product : Product
  CLAWS_ElvLhIBCmdDeg : Outport
  wires:
  Add/1 -> CLAWS_ElvLhIBCmdDeg/1  "REFSI_FD_IN_nmodeElvLhInbdCmd_Deg"
  [CLAWsCommands] -> Bus Selector6/1
  In1/1 -> Add/2
  Bus Selector6/1 -> Product/2
  Product/1 -> Add/1
  [CLAWsOn] -> Product/1

== system Lib_Piccolo/A//C Dynamics/Simulated Piccolo Commands/Subsystem5 ==
  In1 : Inport
  Add : Sum  Inputs=++|
  Bus Selector6 : BusSelector  OutputSignals=REFSI_AC_OUT_nmodeRudLhPylonCmd_Deg
  Product : Product
  CLAWS_RudPylLhCmdDeg : Outport
  wires:
  [CLAWsOn] -> Product/1
  Product/1 -> Add/1
  Bus Selector6/1 -> Product/2  "<REFSI_AC_OUT_nmodeRudLhPylonCmd_Deg>"
  In1/1 -> Add/2
  [CLAWsCommands] -> Bus Selector6/1
  Add/1 -> CLAWS_RudPylLhCmdDeg/1  "REFSI_FD_IN_nmodeRudLhPylonCmd_Deg"

== system Lib_Piccolo/A//C Dynamics/Simulated Piccolo Commands/Subsystem6 ==
  In1 : Inport
  Add : Sum  Inputs=++|
  Bus Selector6 : BusSelector  OutputSignals=REFSI_AC_OUT_nmodeRudLhUTailCmd_Deg
  Product : Product
  CLAWS_RudUTailLhCmdDeg : Outport
  wires:
  Add/1 -> CLAWS_RudUTailLhCmdDeg/1  "REFSI_FD_IN_nmodeRudLhUTailCmd_Deg"
  [CLAWsCommands] -> Bus Selector6/1
  In1/1 -> Add/2
  Bus Selector6/1 -> Product/2  "<REFSI_AC_OUT_nmodeRudLhUTailCmd_Deg>"
  Product/1 -> Add/1
  [CLAWsOn] -> Product/1

== system Lib_Piccolo/A//C Dynamics/Simulated Piccolo Commands/Subsystem7 ==
  In1 : Inport
  Add : Sum  Inputs=++|
  Bus Selector6 : BusSelector  OutputSignals=REFSI_AC_OUT_nmodeElvLhUTailCmd_Deg
  Product : Product
  CLAWS_ElvUTailLhCmdDeg : Outport
  wires:
  [CLAWsOn] -> Product/1
  Product/1 -> Add/1
  Bus Selector6/1 -> Product/2  "<REFSI_AC_OUT_nmodeElvLhUTailCmd_Deg>"
  In1/1 -> Add/2
  [CLAWsCommands] -> Bus Selector6/1
  Add/1 -> CLAWS_ElvUTailLhCmdDeg/1  "REFSI_FD_IN_nmodeElvLhUTailCmd_Deg"

== system Lib_Piccolo/A//C Dynamics/Simulated Piccolo Commands/Subsystem8 ==
  In1 : Inport
  Add : Sum  Inputs=++|
  Bus Selector6 : BusSelector  OutputSignals=REFSI_AC_OUT_nmodeAftFlapCmd_Deg
  Product : Product
  CLAWS_AftFlapCmdDeg : Outport
  wires:
  Add/1 -> CLAWS_AftFlapCmdDeg/1  "REFSI_FD_IN_nmodeAftFlapCmd_Deg"
  [CLAWsCommands] -> Bus Selector6/1
  In1/1 -> Add/2
  Bus Selector6/1 -> Product/2  "<REFSI_AC_OUT_nmodeAftFlapCmd_Deg>"
  Product/1 -> Add/1
  [CLAWsOn] -> Product/1

== system Lib_Piccolo/A//C Dynamics/Simulated Piccolo Commands/Subsystem9 ==
  In1 : Inport
  Add : Sum  Inputs=++|
  Bus Selector6 : BusSelector  OutputSignals=REFSI_AC_OUT_nmodeElvRhUTailCmd_Deg
  Product : Product
  CLAWS_ElvUTailRhCmdDeg : Outport
  wires:
  [CLAWsOn] -> Product/1
  Product/1 -> Add/1
  Bus Selector6/1 -> Product/2  "<REFSI_AC_OUT_nmodeElvRhUTailCmd_Deg>"
  In1/1 -> Add/2
  [CLAWsCommands] -> Bus Selector6/1
  Add/1 -> CLAWS_ElvUTailRhCmdDeg/1  "REFSI_FD_IN_nmodeElvRhUTailCmd_Deg"

== system Lib_Piccolo/A//C Dynamics Full Interface/DLLSimulation/Bus2Vect2 ==
  In1 : Inport
  BusSelector : BusSelector  OutputSignals=REFSI_FD_IN_nmodeRudLhWingCmd_Deg (signal 1),REFSI_FD_IN_nmodeAilLhLowerCmd_Deg (signal 2),REFSI_FD_IN_nmodeAilLhUpperCmd_Deg (signal 3),REFSI_FD_IN_nmodeElvLhOutbdCmd_Deg (signal 4),REFSI_FD_IN_nmodeElvLhInbdCmd_Deg (signal 5),REFSI_FD_IN_nmodeRudLhPylonCmd_Deg (signal 6),REFSI_FD_IN_nmodeRudLhUTailCmd_Deg (signal 7),REFSI_FD_IN_nmodeElvLhUTailCmd_Deg (signal 8),REFSI_FD_IN_nmodeAftFlapCmd_Deg (signal 9),REFSI_FD_IN_nmodeElvRhUTailCmd_Deg (signal 10),REFSI_FD_IN_nmodeRudRhUTailCmd_Deg (signal 11),REFSI_FD_IN_nmodeRudRhPylonCmd_Deg (signal 12),REFSI_FD_IN_nmodeElvRhInbdCmd_Deg (signal 13),REFSI_FD_IN_nmodeElvRhOutbdCmd_Deg (signal 14),REFSI_FD_IN_nmodeAilRhUpperCmd_Deg (signal 15),REFSI_FD_IN_nmodeAilRhLowerCmd_Deg (signal 16),REFSI_FD_IN_nmodeRudRhWingCmd_Deg (signal 17),REFSI_FD_IN_nmodeStabCmd (signal 18),REFSI_FD_IN_nmodeFlapLhOBPosn_Deg (signal 19),REFSI_FD_IN_nmodeFlapLhIBPosn_Deg (signal 20),REFSI_FD_IN_nmodeSlatLhPosn_Deg (signal 21),REFSI_FD_IN_nmodeSlatRhPosn_Deg (signal 22),REFSI_FD_IN_nmodeFlapRhOBPosn_Deg (signal 23),REFSI_FD_IN_nmodeFlapRhIBPosn_Deg (signal 24),REFSI_FD_IN_nmodeTlaLhCmd_Deg (signal 25),REFSI_FD_IN_nmodeTlaLhCmd_Deg (signal 26),EngineLhFuelCut (signal 27),EngineRhFuelCut (signal 28),REFSI_FD_IN_nmodeBrakeCmd (signal 29),REFSI_FD_IN_nmodeNoseGearCmd_Deg (signal 30),REFSI_FD_IN_nmodeSplrLhOutbdCmd_Deg (signal 31),REFSI_FD_IN_nmodeSplrLhInbdCmd_Deg (signal 32),REFSI_FD_IN_nmodeSplrRhInbdCmd_Deg (signal 33),REFSI_FD_IN_nmodeSplrRhOutbdCmd_Deg (signal 34),REFSI_FD_IN_nmodeCgShifterCmd_Ft (signal 35),piccoloInCmd (signal 36),pilotNzCmd_g (signal 37),isControlSurfaceCmdFromSystem (signal 38),nmodeReset (signal 39)
  Mux : Mux  Inputs=39
  Out1 : Outport
  wires:
  In1/1 -> BusSelector/1
  Mux/1 -> Out1/1
